simulink model "Test3D_Balls_in_Box"  (R2024a)
settings: Solver=ode23t  StartTime=0.0  StopTime=20  MaxStep=1e-2  RelTol=1e-4  AbsTol=1e-5  EnableMultiTasking=on
StartFcn:
  | tic;
StopFcn:
  | Elapsed_Sim_Time = toc;
  | disp(['Elapsed Sim Time = ' num2str(Elapsed_Sim_Time)]);
model workspace (MATLAB code in the model file):
  | box.length = 8;
  | box.width = 6;
  | box.height = 4;
  | box.wall_thickness = 0.005;
  | 
  | ball.radius = 0.5;
  | ball.density = 1000;
undefined symbols (not defined in the file or in its folder): X, Y, Z
libraries: sm_lib x23, Contact_Forces_Lib x18, Parts_Lib x3, nesl_utility x1
(part 2 of 2)

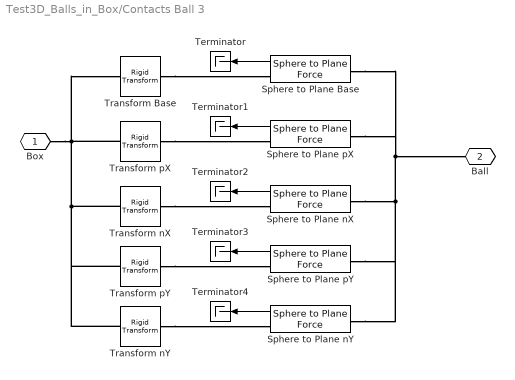
== system Test3D_Balls_in_Box/Contacts Ball 3 ==
  Sphere to Plane Base : Contact_Forces_Lib/3D/Sphere to Plane Force  sphere_rad=ball_rad  plane_lenx=box_l  plane_leny=box_w  plane_depth=box.wall_thickness/2  force_law=Nonlinear  k_contact=1e7  b_contact=1e4  pen_full_damp_F=1e-4  pen_exponent=1  custom_param_1=1  custom_param_2=1  friction_law=None  mu_kinetic=0.5  mu_static=0.7  v_thr=0.001  vis_on=off  vis_opc_en=0  vis_len_plaBz=box.wall_thickness*0.25  vis_clr=[0.9 0.2 0.2]  vis_opc=0.7
  Sphere to Plane nX : Contact_Forces_Lib/3D/Sphere to Plane Force  sphere_rad=ball_rad  plane_lenx=box_h  plane_leny=box_w  plane_depth=box.wall_thickness/2  force_law=Nonlinear  k_contact=1e7  b_contact=1e4  pen_full_damp_F=1e-4  pen_exponent=1  custom_param_1=1  custom_param_2=1  friction_law=None  mu_kinetic=0.5  mu_static=0.7  v_thr=0.001  vis_on=off  vis_opc_en=0  vis_len_plaBz=box.wall_thickness*0.25  vis_clr=[0.9 0.2 0.2]  vis_opc=0.7
  Sphere to Plane nY : Contact_Forces_Lib/3D/Sphere to Plane Force  sphere_rad=ball_rad  plane_lenx=box_l  plane_leny=box_h  plane_depth=box.wall_thickness/2  force_law=Nonlinear  k_contact=1e7  b_contact=1e4  pen_full_damp_F=1e-4  pen_exponent=1  custom_param_1=1  custom_param_2=1  friction_law=None  mu_kinetic=0.5  mu_static=0.7  v_thr=0.001  vis_on=off  vis_opc_en=0  vis_len_plaBz=box.wall_thickness*0.25  vis_clr=[0.9 0.2 0.2]  vis_opc=0.7
  Sphere to Plane pX : Contact_Forces_Lib/3D/Sphere to Plane Force  sphere_rad=ball_rad  plane_lenx=box_h  plane_leny=box_w  plane_depth=box.wall_thickness  force_law=Nonlinear  k_contact=1e7  b_contact=1e4  pen_full_damp_F=1e-4  pen_exponent=1  custom_param_1=1  custom_param_2=1  friction_law=None  mu_kinetic=0.5  mu_static=0.7  v_thr=0.001  vis_on=off  vis_opc_en=0  vis_len_plaBz=box.wall_thickness*0.25  vis_clr=[0.9 0.2 0.2]  vis_opc=0.7
  Sphere to Plane pY : Contact_Forces_Lib/3D/Sphere to Plane Force  sphere_rad=ball_rad  plane_lenx=box_l  plane_leny=box_h  plane_depth=box.wall_thickness/2  force_law=Nonlinear  k_contact=1e7  b_contact=1e4  pen_full_damp_F=1e-4  pen_exponent=1  custom_param_1=1  custom_param_2=1  friction_law=None  mu_kinetic=0.5  mu_static=0.7  v_thr=0.001  vis_on=off  vis_opc_en=0  vis_len_plaBz=box.wall_thickness*0.25  vis_clr=[0.9 0.2 0.2]  vis_opc=0.7
  Terminator{,1..4} (5 alike) : Terminator
  Transform Base : sm_lib/Frames and Transforms/Rigid Transform  RotationMethod=None  FollAlignAxisA=+X  BaseAlignAxisA=+Y  FollAlignAxisB=+Y  BaseAlignAxisB=+Z  RotationStandardAxis=+Z  RotationAngle=0.0  RotationAngleUnits=deg  RotationArbitraryAxis=[0 0 1]  RotationSequenceAxes=FollowerAxes  RotationSequence=XYX  RotationSequenceAngles=[0 0 0]  RotationSequenceAnglesUnits=deg  RotationMatrix=[1 0 0; 0 1 0; 0 0 1]  Quaternion=[1 0 0 0]  TranslationMethod=StandardAxis  TranslationCartesianOffset=[0 0 0]  TranslationCartesianOffsetUnits=m  TranslationStandardAxis=+Z  TranslationStandardOffset=-box_h/2-box.wall_thickness/2  TranslationStandardOffsetUnits=m  TranslationROffset=0  TranslationROffsetUnits=m  TranslationThetaOffset=0  TranslationThetaOffsetUnits=deg  TranslationZOffset=0  TranslationZOffsetUnits=m
  Transform nX : sm_lib/Frames and Transforms/Rigid Transform  RotationMethod=StandardAxis  FollAlignAxisA=+X  BaseAlignAxisA=+Y  FollAlignAxisB=+Y  BaseAlignAxisB=+Z  RotationStandardAxis=+Y  RotationAngle=90.0  RotationAngleUnits=deg  RotationArbitraryAxis=[0 0 1]  RotationSequenceAxes=FollowerAxes  RotationSequence=XYX  RotationSequenceAngles=[0 0 0]  RotationSequenceAnglesUnits=deg  RotationMatrix=[1 0 0; 0 1 0; 0 0 1]  Quaternion=[1 0 0 0]  TranslationMethod=StandardAxis  TranslationCartesianOffset=[0 0 0]  TranslationCartesianOffsetUnits=m  TranslationStandardAxis=-X  TranslationStandardOffset=box_l/2+box.wall_thickness/2  TranslationStandardOffsetUnits=m  TranslationROffset=0  TranslationROffsetUnits=m  TranslationThetaOffset=0  TranslationThetaOffsetUnits=deg  TranslationZOffset=0  TranslationZOffsetUnits=m
  Transform nY : sm_lib/Frames and Transforms/Rigid Transform  RotationMethod=StandardAxis  FollAlignAxisA=+X  BaseAlignAxisA=+Y  FollAlignAxisB=+Y  BaseAlignAxisB=+Z  RotationStandardAxis=-X  RotationAngle=90.0  RotationAngleUnits=deg  RotationArbitraryAxis=[0 0 1]  RotationSequenceAxes=FollowerAxes  RotationSequence=XYX  RotationSequenceAngles=[0 0 0]  RotationSequenceAnglesUnits=deg  RotationMatrix=[1 0 0; 0 1 0; 0 0 1]  Quaternion=[1 0 0 0]  TranslationMethod=StandardAxis  TranslationCartesianOffset=[0 0 0]  TranslationCartesianOffsetUnits=m  TranslationStandardAxis=-Y  TranslationStandardOffset=box_w/2+box.wall_thickness/2  TranslationStandardOffsetUnits=m  TranslationROffset=0  TranslationROffsetUnits=m  TranslationThetaOffset=0  TranslationThetaOffsetUnits=deg  TranslationZOffset=0  TranslationZOffsetUnits=m
  Transform pX : sm_lib/Frames and Transforms/Rigid Transform  RotationMethod=StandardAxis  FollAlignAxisA=+X  BaseAlignAxisA=+Y  FollAlignAxisB=+Y  BaseAlignAxisB=+Z  RotationStandardAxis=-Y  RotationAngle=90.0  RotationAngleUnits=deg  RotationArbitraryAxis=[0 0 1]  RotationSequenceAxes=FollowerAxes  RotationSequence=XYX  RotationSequenceAngles=[0 0 0]  RotationSequenceAnglesUnits=deg  RotationMatrix=[1 0 0; 0 1 0; 0 0 1]  Quaternion=[1 0 0 0]  TranslationMethod=StandardAxis  TranslationCartesianOffset=[0 0 0]  TranslationCartesianOffsetUnits=m  TranslationStandardAxis=+X  TranslationStandardOffset=box_l/2+box.wall_thickness/2  TranslationStandardOffsetUnits=m  TranslationROffset=0  TranslationROffsetUnits=m  TranslationThetaOffset=0  TranslationThetaOffsetUnits=deg  TranslationZOffset=0  TranslationZOffsetUnits=m
  Transform pY : sm_lib/Frames and Transforms/Rigid Transform  RotationMethod=StandardAxis  FollAlignAxisA=+X  BaseAlignAxisA=+Y  FollAlignAxisB=+Y  BaseAlignAxisB=+Z  RotationStandardAxis=+X  RotationAngle=90.0  RotationAngleUnits=deg  RotationArbitraryAxis=[0 0 1]  RotationSequenceAxes=FollowerAxes  RotationSequence=XYX  RotationSequenceAngles=[0 0 0]  RotationSequenceAnglesUnits=deg  RotationMatrix=[1 0 0; 0 1 0; 0 0 1]  Quaternion=[1 0 0 0]  TranslationMethod=StandardAxis  TranslationCartesianOffset=[0 0 0]  TranslationCartesianOffsetUnits=m  TranslationStandardAxis=+Y  TranslationStandardOffset=box_w/2+box.wall_thickness/2  TranslationStandardOffsetUnits=m  TranslationROffset=0  TranslationROffsetUnits=m  TranslationThetaOffset=0  TranslationThetaOffsetUnits=deg  TranslationZOffset=0  TranslationZOffsetUnits=m
  Box : PMIOPort  Side=Left
  Ball : PMIOPort  Port=2  Side=Right
  wires:
  Sphere to Plane pX/1 -> Terminator1/1
  Sphere to Plane nX/1 -> Terminator2/1
  Sphere to Plane pY/1 -> Terminator3/1
  Sphere to Plane nY/1 -> Terminator4/1
  Sphere to Plane Base/1 -> Terminator/1
  connections:
  Transform Base/RConn1 -- Sphere to Plane Base/RConn1
  Sphere to Plane nX/LConn1 -- Sphere to Plane pX/LConn1 -- Sphere to Plane Base/LConn1 -- Ball/RConn1 -- Sphere to Plane nY/LConn1 -- Sphere to Plane pY/LConn1
  Box/RConn1 -- Transform pX/LConn1 -- Transform Base/LConn1 -- Transform nX/LConn1 -- Transform pY/LConn1 -- Transform nY/LConn1
  Transform pX/RConn1 -- Sphere to Plane pX/RConn1
  Transform nX/RConn1 -- Sphere to Plane nX/RConn1
  Transform pY/RConn1 -- Sphere to Plane pY/RConn1
  Transform nY/RConn1 -- Sphere to Plane nY/RConn1
